simulink model "bchc"  (Simulink 7.4)
settings: Solver=ode23tb  StartTime=0.0  StopTime=0.01  MaxStep=5e-6  RelTol=1e-3
libraries: powerlib x17, simulink x1
settings Model: Creator=kAnnanvalar  LastModifiedBy=kAnnanvalar

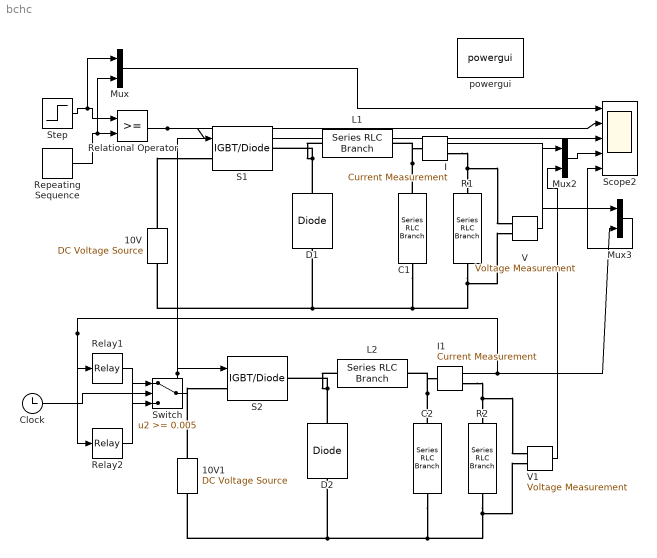
== system bchc ==
  10V : powerlib/Electrical Sources/DC Voltage Source  DialogController=POWERSYS.PowerSysDialog  SystemSampleTime=-1  Amplitude=10  Measurements=None
  10V1 : powerlib/Electrical Sources/DC Voltage Source  DialogController=POWERSYS.PowerSysDialog  SystemSampleTime=-1  Amplitude=10  Measurements=None
  C1 : powerlib/Elements/Series RLC Branch  DialogController=POWERSYS.PowerSysDialog  PhysicalDomain=powersysdomain  SubClassName=unknown  LeftPortType=p1  RightPortType=p1  LConnTagsString=__new0  RConnTagsString=__new0  BranchType=C  Resistance=1  Inductance=1e-3  SetiL0=off  InitialCurrent=0  Capacitance=0.4e-6  Setx0=off  InitialVoltage=0  Measurements=None
  C2 : powerlib/Elements/Series RLC Branch  DialogController=POWERSYS.PowerSysDialog  PhysicalDomain=powersysdomain  SubClassName=unknown  LeftPortType=p1  RightPortType=p1  LConnTagsString=__new0  RConnTagsString=__new0  BranchType=C  Resistance=1  Inductance=1e-3  SetiL0=off  InitialCurrent=0  Capacitance=0.4e-6  Setx0=off  InitialVoltage=0  Measurements=None
  Clock : Clock
      settings: Decimation=10
  D1 : powerlib/Power Electronics/Diode  DialogController=POWERSYS.PowerSysDialog  SystemSampleTime=-1  Ron=0.001  Lon=0  Vf=0.8  IC=0  UseSnubber=off  Rs=500  Cs=250e-9  Measurements=off
  D2 : powerlib/Power Electronics/Diode  DialogController=POWERSYS.PowerSysDialog  SystemSampleTime=-1  Ron=0.001  Lon=0  Vf=0.8  IC=0  UseSnubber=off  Rs=500  Cs=250e-9  Measurements=off
  I : powerlib/Measurements/Current Measurement  DialogController=POWERSYS.PowerSysDialog  SystemSampleTime=-1  PhasorSimulation=off  OutputType=Complex  PSBequivalent=0
  I1 : powerlib/Measurements/Current Measurement  DialogController=POWERSYS.PowerSysDialog  SystemSampleTime=-1  PhasorSimulation=off  OutputType=Complex  PSBequivalent=0
  L1 : powerlib/Elements/Series RLC Branch  DialogController=POWERSYS.PowerSysDialog  PhysicalDomain=powersysdomain  SubClassName=unknown  LeftPortType=p1  RightPortType=p1  LConnTagsString=__new0  RConnTagsString=__new0  BranchType=L  Resistance=50  Inductance=5.83e-3  SetiL0=off  InitialCurrent=0  Capacitance=1e-6  Setx0=off  InitialVoltage=0  Measurements=None
  L2 : powerlib/Elements/Series RLC Branch  DialogController=POWERSYS.PowerSysDialog  PhysicalDomain=powersysdomain  SubClassName=unknown  LeftPortType=p1  RightPortType=p1  LConnTagsString=__new0  RConnTagsString=__new0  BranchType=L  Resistance=50  Inductance=5.83e-3  SetiL0=off  InitialCurrent=0  Capacitance=1e-6  Setx0=off  InitialVoltage=0  Measurements=None
  Mux : Mux  Inputs=2
  Mux2 : Mux  Inputs=2
  Mux3 : Mux  Inputs=2
  R1 : powerlib/Elements/Series RLC Branch  DialogController=POWERSYS.PowerSysDialog  PhysicalDomain=powersysdomain  SubClassName=unknown  LeftPortType=p1  RightPortType=p1  LConnTagsString=__new0  RConnTagsString=__new0  BranchType=R  Resistance=500  Inductance=0.1  SetiL0=off  InitialCurrent=0  Capacitance=1e-6  Setx0=off  InitialVoltage=0  Measurements=None
  R2 : powerlib/Elements/Series RLC Branch  DialogController=POWERSYS.PowerSysDialog  PhysicalDomain=powersysdomain  SubClassName=unknown  LeftPortType=p1  RightPortType=p1  LConnTagsString=__new0  RConnTagsString=__new0  BranchType=R  Resistance=500  Inductance=0.1  SetiL0=off  InitialCurrent=0  Capacitance=1e-6  Setx0=off  InitialVoltage=0  Measurements=None
  Relational Operator : RelationalOperator  LogicOutDataTypeMode=boolean  LogicDataType=fixdt(0, 8)  OutDataTypeStr=boolean
  Relay1 : Relay  OnSwitchValue=3.75e-3  OffSwitchValue=3.65e-3  OnOutputValue=0  OffOutputValue=1  OutDataType=fixdt(1, 16)  OutScaling=2^0
  Relay2 : Relay  OnSwitchValue=0.0155  OffSwitchValue=0.0154  OnOutputValue=0  OffOutputValue=1  OutDataType=fixdt(1, 16)  OutScaling=2^0
  Repeating Sequence : simulink/Sources/Repeating Sequence  SystemSampleTime=-1  rep_seq_t=[0 1/25e3]  rep_seq_y=[0 1]
  S1 : powerlib/Power Electronics/IGBT//Diode  DialogController=POWERSYS.PowerSysDialog  SystemSampleTime=-1  Ron=1e-3  Rs=1e5  Cs=inf  Measurements=off
  S2 : powerlib/Power Electronics/IGBT//Diode  DialogController=POWERSYS.PowerSysDialog  SystemSampleTime=-1  Ron=1e-3  Rs=1e5  Cs=inf  Measurements=off
  Scope2 : Scope  NumInputPorts=5
      settings: YMin=0~0~-10~5.55112e-017~-5  YMax=1~1~110~1.4~5  MaxDataPoints=5000000
  Step : Step  Time=0.005  Before=0.2  After=0.8  SampleTime=0
  Switch : Switch  Threshold=0.005  OutDataType=fixdt(1, 16)  OutScaling=2^0
  V : powerlib/Measurements/Voltage Measurement  DialogController=POWERSYS.PowerSysDialog  SystemSampleTime=-1  PhasorSimulation=off  OutputType=Complex  PSBequivalent=0
  V1 : powerlib/Measurements/Voltage Measurement  DialogController=POWERSYS.PowerSysDialog  SystemSampleTime=-1  PhasorSimulation=off  OutputType=Complex  PSBequivalent=0
  powergui : powerlib/powergui  Priority=1  SystemSampleTime=-1  SimulationMode=Continuous  SampleTime=50e-6  frequency=60  SPID=off  DisableSnubberDevices=off  DisableRonSwitches=off  DisableVfSwitches=off  SwTol=0  Interpol=off  frequencyindice=0  echomessages=off  HookPort=off  DisplayEquations=off  FunctionMessages=off  EnableUseOfTLC=off  x0status=blocks  RestoreLinks=warning  Frange=[0:2:500]  Ylog=off  Xlog=on  ShowGrid=off  save=off  variable=ZData  ZoomFFT=on  StartTime=0.0  cycles=1  DisplayStyle=1  fundamental=60  FreqAxis=off  MaxFrequency=1000  frequencyindicesteady=1  RmsSteady=1  display=off  Ts=0  methode=off
  wires:
  Step/1 -> Relational Operator/1, Mux/1
  Repeating Sequence/1 -> Relational Operator/2, Mux/2
  Relational Operator/1 -> Scope2/2, S1/1
  Mux/1 -> Scope2/1
  V/1 -> Mux2/1
  V1/1 -> Mux2/2
  I/1 -> Mux3/1
  I1/1 -> Mux3/2, Relay1/1, Relay2/1
  Switch/1 -> S2/1, Scope2/3
  Mux2/1 -> Scope2/4
  Mux3/1 -> Scope2/5
  Clock/1 -> Switch/2
  Relay2/1 -> Switch/1
  Relay1/1 -> Switch/3
  connections:
  10V/RConn1 -- S1/LConn1
  C1/LConn1 -- I/LConn1 -- L1/LConn1
  R1/RConn1 -- V/LConn2 -- 10V/LConn1 -- D1/LConn1 -- C1/RConn1
  I/RConn1 -- R1/LConn1 -- V/LConn1
  D1/RConn1 -- S1/RConn1 -- L1/RConn1
  C2/LConn1 -- L2/LConn1 -- I1/LConn1
  R2/RConn1 -- V1/LConn2 -- C2/RConn1 -- D2/LConn1 -- 10V1/LConn1
  I1/RConn1 -- V1/LConn1 -- R2/LConn1
  D2/RConn1 -- L2/RConn1 -- S2/RConn1
  10V1/RConn1 -- S2/LConn1
